simulink model "fdir_simulink"  (R2026b)
settings: Solver=VariableStepAuto
InitFcn:
  | init_fdir
settings Model: Creator=aditi  LastModifiedBy=aditi

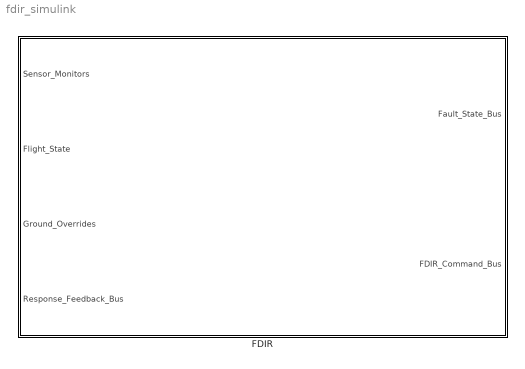
== system fdir_simulink ==
  FDIR : Subsystem

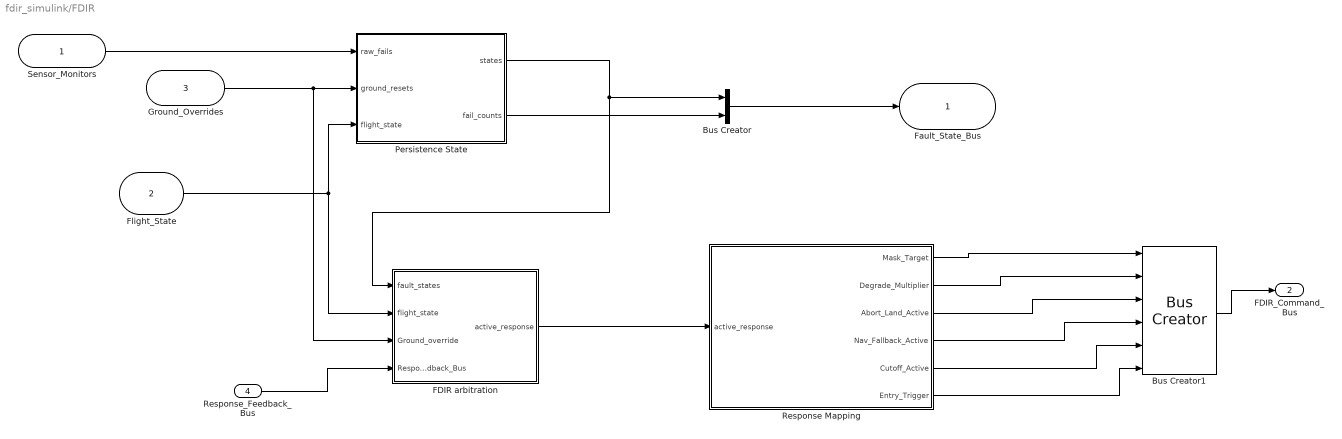
== system fdir_simulink/FDIR ==
  Sensor_Monitors : Inport
  Flight_State : Inport  Port=2
  Ground_Overrides : Inport  Port=3
  Response_Feedback_Bus : Inport  Port=4  OutDataTypeStr=Bus: Response_Feedback_Bus
  Bus Creator : BusCreator  Inputs=2
  Bus Creator1 : BusCreator  Inputs=6  OutDataTypeStr=Bus: FDIR_Command_Bus
  FDIR arbitration : MATLAB Function  TreatAsAtomicUnit=on  SystemSampleTime=0.01
  Persistence State : MATLAB Function  TreatAsAtomicUnit=on  SystemSampleTime=0.01
  Response Mapping : MATLAB Function  TreatAsAtomicUnit=on  SystemSampleTime=0.01
  Fault_State_Bus : Outport
  FDIR_Command_Bus : Outport  Port=2
  wires:
  Sensor_Monitors/1 -> Persistence State/1(raw_fails)
  Persistence State/1(states) -> FDIR arbitration/1(fault_states), Bus Creator/1
  Persistence State/2(fail_counts) -> Bus Creator/2
  Bus Creator/1 -> Fault_State_Bus/1
  FDIR arbitration/1(active_response) -> Response Mapping/1(active_response)
  Ground_Overrides/1 -> FDIR arbitration/3(Ground_override), Persistence State/2(ground_resets)
  Flight_State/1 -> Persistence State/3(flight_state), FDIR arbitration/2(flight_state)
  Response Mapping/1(Mask_Target) -> Bus Creator1/1
  Response Mapping/2(Degrade_Multiplier) -> Bus Creator1/2
  Response Mapping/3(Abort_Land_Active) -> Bus Creator1/3
  Response Mapping/4(Nav_Fallback_Active) -> Bus Creator1/4
  Response Mapping/5(Cutoff_Active) -> Bus Creator1/5
  Bus Creator1/1 -> FDIR_Command_Bus/1
  Response Mapping/6(Entry_Trigger) -> Bus Creator1/6
  Response_Feedback_Bus/1 -> FDIR arbitration/4(Response_Feedback_Bus)

== matlab function fdir_simulink/FDIR/FDIR arbitration ==
  data: fault_states input; active_response output; flight_state input; Ground_override input; Response_Feedback_Bus input; fault_config parameter
function active_response = fdir_arbitration(fault_states, flight_state, Ground_override, Response_Feedback_Bus, fault_config)
% Persistent state across simulation steps
persistent current_response;

% Initialize on first simulation step with explicit uint8 type
if isempty(current_response)
    current_response = uint8(0); % Start at R0 (Nominal)
end

% Define Flight Phase Enums for context
LANDED_PHASE = uint8(5); % Example: 5 represents the safe LANDED state

% Ground Override / Post-Landing Reset Policy:
% Allow clearing response level ONLY if the vehicle is safely landed 
% AND a valid ground override command is given.
if Ground_override && (flight_state == LANDED_PHASE)
    current_response = uint8(0);
    active_response = current_response;
    return;
end

max_requested = uint8(0);

% Loop through each independent fault state in the vector
for i = 1:length(fault_states)
    sensor_state = fault_states(i);

    % Evaluate response level only if the fault is latched (state == 2)
    if sensor_state == uint8(2)
        % Evaluate response level only if the fault is latched (state == 2)
        if sensor_state == uint8(2)
            % Dynamic lookup from table-driven configuration traceable to CoDR
            req = fault_config(i).Response_Tier;
        else
            req = uint8(0); % Nominal for this monitor
        end
    else
        req = uint8(0); % Nominal for this monitor
    end

    % Max-Severity Selection: Find the highest response tier required across all monitors
    if req > max_requested
        max_requested = req;
    end
end

% Enforce Monotonic Escalation Latch
% The vehicle response can only step UP during flight. 
% It ignores transient drops or lower fault requests once escalated.
if max_requested > current_response
    current_response = max_requested;
end

active_response = current_response;
end

== matlab function fdir_simulink/FDIR/Persistence State ==
  data: raw_fails input; states output; fail_counts output; ground_resets input; flight_state input; fault_config parameter
function [states, fail_counts] = fdir_persistence_vector(raw_fails, ground_resets, flight_state, fault_config)
% Persistent matrices across simulation steps (Size: [Num_Faults, M])
persistent history;     
persistent states_vec;  

% Configuration parameters
M = 10; % Window size (last 10 frames)
N = 4;  % Failure threshold (4 out of 10)

% Define active flight phases (e.g., 2=Ascent, 3=Hover, 4=Descent)
active_phases = [2, 3, 4]; 

num_faults = length(raw_fails);

% Initialize on first simulation step
if isempty(history)
    history = false(num_faults, M);
    states_vec = zeros(num_faults, 1); % 0: INACTIVE, 1: PENDING, 2: LATCHED
end

fail_counts = zeros(num_faults, 1);

% Loop through each individual fault monitor independently
for i = 1:num_faults

    % Handle individual Ground Reset for this specific fault ID
    if ground_resets(i)
        history(i, :) = false(1, M);
        states_vec(i) = 0;
        fail_counts(i) = 0;
        continue;
    end

    % Phase Mask Check: Pause evaluation if outside active phases
    if ~ismember(flight_state, active_phases)
        if states_vec(i) ~= 2
            history(i, :) = false(1, M);
            states_vec(i) = 0;
        end
        fail_counts(i) = sum(history(i, :));
        continue;
    end

    % If already latched, hold state
    if states_vec(i) == 2
        fail_counts(i) = sum(history(i, :));
        continue;
    end

    % Shift history window and record latest sample for fault i
    history(i, :) = [history(i, 2:end), logical(raw_fails(i))];

    % Count total failures in window for fault i
    fail_counts(i) = sum(history(i, :));

    % State Machine Transitions per fault ID
    switch states_vec(i)
        case 0 % INACTIVE
            if raw_fails(i)
                states_vec(i) = 1; % Transition to PENDING
            end

        case 1 % PENDING
            if fail_counts(i) >= N
                states_vec(i) = 2; % Transition to LATCHED
            elseif fail_counts(i) == 0
                states_vec(i) = 0; % Return to INACTIVE
            end

        case 2 % LATCHED
            states_vec(i) = 2;
    end
end

states = states_vec;
end

== matlab function fdir_simulink/FDIR/Response Mapping ==
  data: active_response input; Mask_Target output; Degrade_Multiplier output; Abort_Land_Active output; Nav_Fallback_Active output; Cutoff_Active output; Entry_Trigger output; fault_config parameter
function [Mask_Target, Degrade_Multiplier, Abort_Land_Active, Nav_Fallback_Active, Cutoff_Active, Entry_Trigger] = response_mapping(active_response, fault_config)

% Enforce strict uint8 type for code generation
active_response = uint8(active_response);

% Persistent memory to track state transitions
persistent prev_response;
if isempty(prev_response)
    prev_response = uint8(0);
end

% Detect if we just entered a new higher response tier this frame (Edge-Triggered)
Entry_Trigger = logical(active_response ~= prev_response);

% Initialize outputs to nominal defaults with explicit types
Mask_Target         = uint8(0);     
Degrade_Multiplier  = double(1.0);   
Abort_Land_Active   = logical(false); 
Nav_Fallback_Active = logical(false); 
Cutoff_Active       = logical(false); 

% Map active response level to targeted GNC commands
switch active_response
    case uint8(0)
        % R0: Nominal
        Mask_Target        = uint8(0);
        Degrade_Multiplier = double(1.0);
    case uint8(1)
        % R1: Degrade & Mask
        Mask_Target        = uint8(2);   
        Degrade_Multiplier = double(2.5); 
    case uint8(2)
        % R2: Abort to Land
        Abort_Land_Active = logical(true);
    case uint8(3)
        % R3: Navigation-Degraded Abort
        Abort_Land_Active   = logical(true);
        Nav_Fallback_Active = logical(true); 
    case uint8(4)
        % R4: Cutoff & Safing
        Cutoff_Active = logical(true);     
    otherwise
        % Fail-safe default
        Cutoff_Active = logical(true);
end

% Update persistent tracker for the next frame
prev_response = active_response;
end
